simulink subsystem "HEVPowerSplitControl_refsub"  (R2023a)
settings: Solver=VariableStepAuto  StartTime=0.0  StopTime=10.0  RelTol=1e-3
undefined symbols (not defined in the file or in its folder): DiscIntNeverNeededParam, hevcontrol, initial
libraries: simulink x5
settings Model: DefaultTestHarness=HEVPowerSplitControl_refsub_Harness1  Creator=isaacito  LastModifiedBy=isaacito
settings SolverCC: AlgebraicLoopSolver=TrustRegion
settings OptimizationCC: ReuseModelBlockBuffer=off
settings DebuggingCC: UnconnectedInputMsg=warning  UnconnectedOutputMsg=warning  UnconnectedLineMsg=warning
settings ModelReferenceCC: EnableRefExpFcnMdlSchedulingChecks=on
settings RTWCC: DLArmComputeVersion=19.05

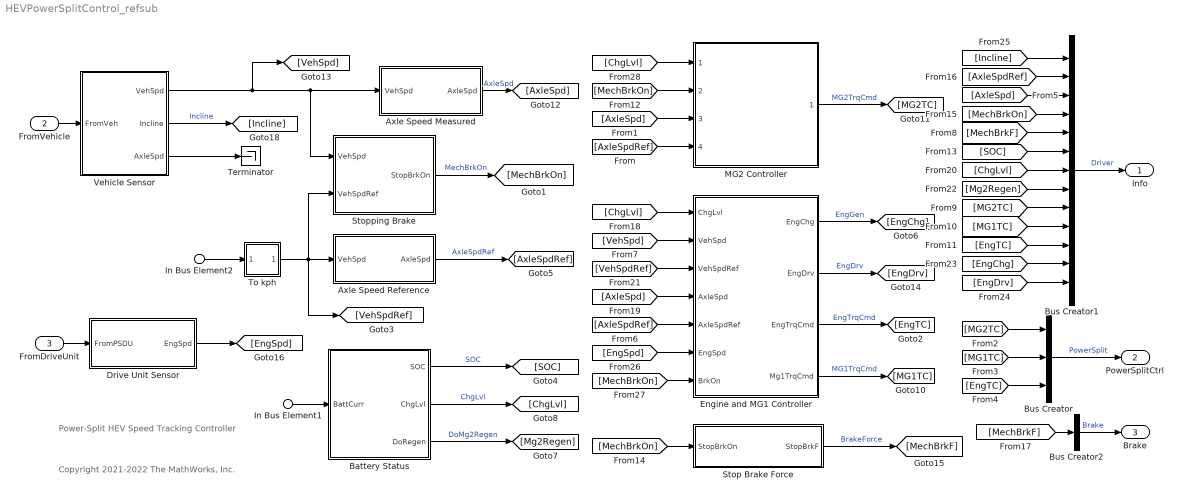
== system HEVPowerSplitControl_refsub ==
  note: Power-Split HEV
      | Speed Tracking Controller
  note: Copyright 2021-2022 The MathWorks, Inc.
  In Bus Element1 : Inport  PortName=FromBattery  Element=Current
  FromVehicle : Inport  Port=2
  FromDriveUnit : Inport  Port=3
  In Bus Element2 : Inport  Port=4  PortName=FromDrvPattern  Element=VehSpdRef
      settings: AttributesFormatString=%<Unit>
  Axle Speed Measured : Subsystem  mask(Vehicle Speed to Axle Speed){Value=hevcontrol.tireRadius_m}
      mask prompts: Value "Tire Rolling Radius [m]"
      mask help: Given longitudinal vehicle speed, this block computes the axle rotational speed.
      mask TypeOptions Value: Tire Rolling Radius (m)/Value
  Axle Speed Reference : Subsystem  mask(Vehicle Speed to Axle Speed){Value=hevcontrol.tireRadius_m}
      mask prompts: Value "Tire Rolling Radius [m]"
      mask help: Given longitudinal vehicle speed, this block computes the axle rotational speed.
      mask TypeOptions Value: Tire Rolling Radius (m)/Value
  Battery Status : Subsystem  mask(Battery Status){capacity_kWh=hevcontrol.hvbattNominalCapacity_kWh, voltagePerCell_V=hevcontrol.hvbattVoltagePerCell_V, initial_SOC_pct=initial.controllerHVBattSOC_pct, SocHigh=hevcontrol.hvbattSocHighMid_pct, SocLow=hevcontrol.hvbattSocMidLow_pct, SocEmpty=hevcontrol.hvbattSocLowEmpty_pct}
      mask prompts: capacity_kWh "Battery Capacity [kW*hr]"; voltagePerCell_V "Voltage per cell [V]"; initial_SOC_pct "Initial SOC [%]"; SocHigh "SOC High-Mid Threshold [%]"; SocLow "SOC Mid-Low Threshold [%]"; SocEmpty "SOC Low-Empty Threshold [%]"
      mask help:
      | Battery current input assumes that the negative (positive) value current means consuming (charging) electric power from (to) the battery.
      |
      | SOC outport outputs the state of charge of the battery in %.
      |
      | ChgLvl outport outputs the charge levels 0 (empty), 1 (low), 2 (mid), or 3 (high). Specify thresholds in SOC Threshold parameters.
      |
      | DoRegen outport outputs true for empty/low/mid battery charge level and false for high. Use this signal to avoid overcharging the battery.
      mask init:
      | if initial_SOC_pct > SocHigh
      |   initialChgLvl = 3;
      | elseif initial_SOC_pct < SocEmpty
      |   initialChgLvl = 0;
      | elseif initial_SOC_pct > SocLow
      |   initialChgLvl = 2;
      | else
      |   initialChgLvl = 1;
      | end
      mask TypeOptions capacity_kWh: SOC Estimation/capacity_kWh
      mask TypeOptions voltagePerCell_V: SOC Estimation/voltagePerCell_V
      mask TypeOptions initial_SOC_pct: SOC Estimation/initial_SOC_pct
      mask DialogControl Container2 Prompt: Parameters
  Bus Creator : BusCreator  Inputs=3
  Bus Creator1 : BusCreator  Inputs=13
  Bus Creator2 : BusCreator  Inputs=1
  Drive Unit Sensor : Subsystem
  Engine and MG1 Controller : Subsystem
  MG2 Controller : Subsystem  ReferencedSubsystem=MG2Controller_HEVPowerSplit_refsub
  Stop Brake Force : Subsystem
  Stopping Brake : Subsystem
  Terminator : Terminator
  To kph : Subsystem
  Vehicle Sensor : Subsystem
  Info : Outport
  PowerSplitCtrl : Outport  Port=2
  Brake : Outport  Port=3
  wires:
  Vehicle Sensor/3(AxleSpd) -> Terminator/1
  In Bus Element2/1 -> To kph/1(In1)
  FromVehicle/1 -> Vehicle Sensor/1(FromVeh)
  Vehicle Sensor/1(VehSpd) -> [VehSpd], Axle Speed Measured/1(VehSpd), Stopping Brake/1(VehSpd)
  Battery Status/1(SOC) -> [SOC]  "SOC"
  [SOC] -> Bus Creator1/6
  [Mg2Regen] -> Bus Creator1/8
  [ChgLvl] -> Bus Creator1/7
  [MechBrkOn] -> Bus Creator1/4
  [AxleSpd] -> Bus Creator1/3
  Engine and MG1 Controller/4(Mg1TrqCmd) -> [MG1TC]  "MG1TrqCmd"
  [VehSpdRef] -> Engine and MG1 Controller/3(VehSpdRef)
  [AxleSpdRef] -> Engine and MG1 Controller/5(AxleSpdRef)
  [AxleSpd] -> Engine and MG1 Controller/4(AxleSpd)
  [AxleSpdRef] -> Bus Creator1/2
  Bus Creator1/1 -> Info/1  "Driver"
  [MG1TC] -> Bus Creator1/10
  [MG2TC] -> Bus Creator1/9
  [MechBrkF] -> Bus Creator1/5
  [EngTC] -> Bus Creator1/11
  [VehSpd] -> Engine and MG1 Controller/2(VehSpd)
  Battery Status/3(DoRegen) -> [Mg2Regen]  "DoMg2Regen"
  Battery Status/2(ChgLvl) -> [ChgLvl]  "ChgLvl"
  Engine and MG1 Controller/3(EngTrqCmd) -> [EngTC]  "EngTrqCmd"
  [ChgLvl] -> Engine and MG1 Controller/1(ChgLvl)
  [EngTC] -> Bus Creator/3
  [MG1TC] -> Bus Creator/2
  [MG2TC] -> Bus Creator/1
  Bus Creator/1 -> PowerSplitCtrl/1  "PowerSplit"
  Axle Speed Reference/1(AxleSpd) -> [AxleSpdRef]  "AxleSpdRef"
  [MechBrkF] -> Bus Creator2/1
  Bus Creator2/1 -> Brake/1  "Brake"
  In Bus Element1/1 -> Battery Status/1(BattCurr)
  Engine and MG1 Controller/1(EngChg) -> [EngChg]  "EngGen"
  Engine and MG1 Controller/2(EngDrv) -> [EngDrv]  "EngDrv"
  [EngChg] -> Bus Creator1/12
  [EngDrv] -> Bus Creator1/13
  [EngSpd] -> Engine and MG1 Controller/6(EngSpd)
  [MechBrkOn] -> Engine and MG1 Controller/7(BrkOn)
  FromDriveUnit/1 -> Drive Unit Sensor/1(FromPSDU)
  Drive Unit Sensor/1(EngSpd) -> [EngSpd]
  [MechBrkOn] -> MG2 Controller/2
  [AxleSpd] -> MG2 Controller/3
  [AxleSpdRef] -> MG2 Controller/4
  [MechBrkOn] -> Stop Brake Force/1(StopBrkOn)
  Vehicle Sensor/2(Incline) -> [Incline]  "Incline"
  MG2 Controller/1 -> [MG2TC]  "MG2TrqCmd"
  Stopping Brake/1(StopBrkOn) -> [MechBrkOn]  "MechBrkOn"
  Stop Brake Force/1(StopBrkF) -> [MechBrkF]  "BrakeForce"
  [Incline] -> Bus Creator1/1
  [ChgLvl] -> MG2 Controller/1
  To kph/1(Out1) -> Axle Speed Reference/1(VehSpd), [VehSpdRef], Stopping Brake/2(VehSpdRef)
  Axle Speed Measured/1(AxleSpd) -> [AxleSpd]  "AxleSpd"

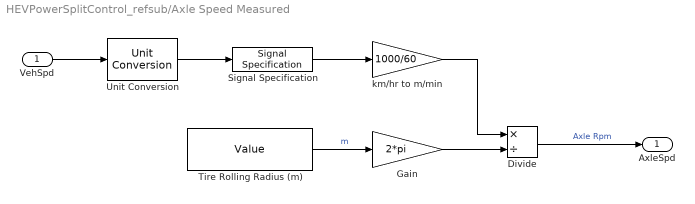
== system HEVPowerSplitControl_refsub/Axle Speed Measured ==
  VehSpd : Inport
      settings: AttributesFormatString=%<Unit>
  Divide : Product  Inputs=*/
  Gain : Gain  Gain=2*pi
  Signal Specification : SignalSpecification  Unit=km/hr
  Tire Rolling Radius (m) : Constant  Value=Value
  Unit Conversion : UnitConversion
  km/hr to m/min : Gain  Gain=1000/60
  AxleSpd : Outport  Unit=rpm  VectorParamsAs1DForOutWhenUnconnected=off
      settings: AttributesFormatString=%<Unit>
  wires:
  km/hr to m/min/1 -> Divide/1
  Signal Specification/1 -> km/hr to m/min/1
  VehSpd/1 -> Unit Conversion/1
  Unit Conversion/1 -> Signal Specification/1
  Divide/1 -> AxleSpd/1  "Axle Rpm"
  Gain/1 -> Divide/2
  Tire Rolling Radius (m)/1 -> Gain/1  "m"

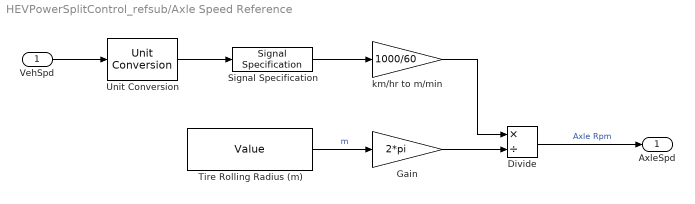
== system HEVPowerSplitControl_refsub/Axle Speed Reference ==
  VehSpd : Inport
      settings: AttributesFormatString=%<Unit>
  Divide : Product  Inputs=*/
  Gain : Gain  Gain=2*pi
  Signal Specification : SignalSpecification  Unit=km/hr
  Tire Rolling Radius (m) : Constant  Value=Value
  Unit Conversion : UnitConversion
  km/hr to m/min : Gain  Gain=1000/60
  AxleSpd : Outport  Unit=rpm  VectorParamsAs1DForOutWhenUnconnected=off
      settings: AttributesFormatString=%<Unit>
  wires:
  km/hr to m/min/1 -> Divide/1
  Signal Specification/1 -> km/hr to m/min/1
  VehSpd/1 -> Unit Conversion/1
  Unit Conversion/1 -> Signal Specification/1
  Divide/1 -> AxleSpd/1  "Axle Rpm"
  Gain/1 -> Divide/2
  Tire Rolling Radius (m)/1 -> Gain/1  "m"

== system HEVPowerSplitControl_refsub/Battery Status ==
  BattCurr : Inport
  Initial Charge Level : InitialCondition  Value=initialChgLvl
  SOC Based States : Stateflow chart  TreatAsAtomicUnit=on
      settings: PortSchema="{\"entries\":[{\"content\":{\"sides\":[{\"content\":{\"connectorIds\":[\"In1\"]},\"type\":\"ConnectorPlacement.EquallySpacedRectSide\",\"uuid\":\"6842a8e0-1533-443f-9239-a32cee073609\"},{\"content\":{\"connectorIds\":[\"Out2\",\"Out1\"],\"side\":\"RIGHT\"},\"type\":\"ConnectorPlacement.EquallySpacedRectSide\",\"uuid\":\"4d5668fa-96aa-414a-86e2-97093b53d80f\"},{\"content\":{\"connectorIds\":[],\"side\":\"TOP\"},\"type\":\"ConnectorPlacement.EquallySpacedRectSide\",\"uuid\":\"b14b12e5-8ddb-4090-8868-1deded7232d1\"},{\"content\":{\"connectorIds\":[],\"side\":\"HIDDEN\"},\"type\":\"ConnectorPlacement.EquallySpacedRectSide\",\"uuid\":\"15641086-7bcd-4523-b266-ad823dacae84\"}]},\"type\":\"ConnectorPlacement.EquallySpacedConnector\",\"uuid\":\"9c75feda-b5f3-44ec-8ad2-652491ceb2eb\"}],\"packageUris\":[\"http://schema.mathworks.com/mf0/Connector/R2020b\"],\"version\":\"1.0\"}"
  SOC Estimation : Subsystem  mask(Battery State-of-Charge Estimation){capacity_kWh=capacity_kWh, voltagePerCell_V=voltagePerCell_V, initial_SOC_pct=initial_SOC_pct}
      mask prompts: capacity_kWh "Battery Capacity [kW*hr]"; voltagePerCell_V "Voltage per cell [V]"; initial_SOC_pct "Initial SOC [%]"
      mask help: Battery current input assumes that the negative value current meas consuming electric power from the battery.
      mask TypeOptions capacity_kWh: Capacity (kW*hr)/Value
      mask TypeOptions voltagePerCell_V: Voltage per Cell (V)/Value
      mask TypeOptions initial_SOC_pct: Initial SOC (%)/Value
  SOC : Outport
  ChgLvl : Outport  Port=2
  DoRegen : Outport  Port=3
  wires:
  Initial Charge Level/1 -> ChgLvl/1
  BattCurr/1 -> SOC Estimation/1(BattCurr)
  SOC Based States/2(BatteryChargeLevel) -> Initial Charge Level/1
  SOC Based States/1(DoRegen) -> DoRegen/1
  SOC Estimation/1(SOC) -> SOC Based States/1(SOC), SOC/1  "SOC"

== system HEVPowerSplitControl_refsub/Drive Unit Sensor ==
  FromPSDU : Inport
  Bus Selector : BusSelector  OutputSignals=eng  OutputAsBus=on
  Bus Selector2 : BusSelector  OutputSignals=EngSpd
  Transfer Fcn : TransferFcn  Denominator=[0.01 1]
  EngSpd : Outport  Unit=rpm
      settings: AttributesFormatString=%<Unit>
  wires:
  Bus Selector/1 -> Bus Selector2/1
  Transfer Fcn/1 -> EngSpd/1
  FromPSDU/1 -> Bus Selector/1
  Bus Selector2/1 -> Transfer Fcn/1  "<EngSpd>"

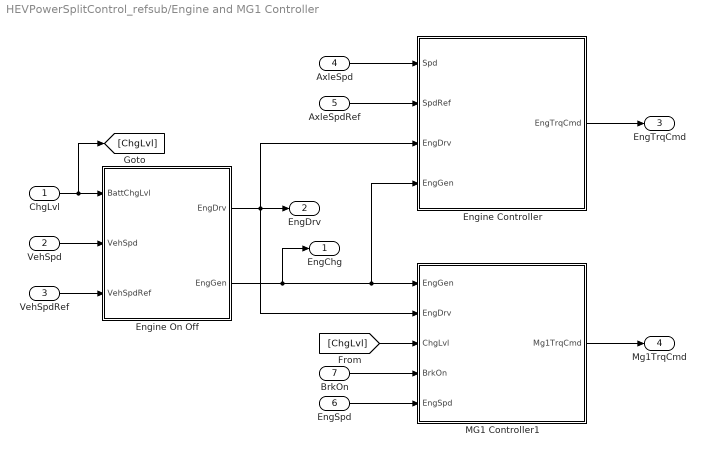
== system HEVPowerSplitControl_refsub/Engine and MG1 Controller ==
  ChgLvl : Inport
  VehSpd : Inport  Port=2  Unit=km/hr
      settings: AttributesFormatString=%<Unit>
  VehSpdRef : Inport  Port=3  Unit=km/hr
      settings: AttributesFormatString=%<Unit>
  AxleSpd : Inport  Port=4  Unit=rpm
      settings: AttributesFormatString=%<Unit>
  AxleSpdRef : Inport  Port=5  Unit=rpm
      settings: AttributesFormatString=%<Unit>
  EngSpd : Inport  Port=6  Unit=rpm
      settings: AttributesFormatString=%<Unit>
  BrkOn : Inport  Port=7
  Engine Controller : Subsystem
  Engine On Off : Stateflow chart  TreatAsAtomicUnit=on
  MG1 Controller1 : Subsystem
  EngChg : Outport
  EngDrv : Outport  Port=2
  EngTrqCmd : Outport  Port=3  Unit=N*m
      settings: AttributesFormatString=%<Unit>
  Mg1TrqCmd : Outport  Port=4  Unit=N*m
      settings: AttributesFormatString=%<Unit>
  wires:
  VehSpd/1 -> Engine On Off/2(VehSpd)
  ChgLvl/1 -> [ChgLvl], Engine On Off/1(BattChgLvl)
  VehSpdRef/1 -> Engine On Off/3(VehSpdRef)
  AxleSpd/1 -> Engine Controller/1(Spd)
  AxleSpdRef/1 -> Engine Controller/2(SpdRef)
  Engine Controller/1(EngTrqCmd) -> EngTrqCmd/1
  BrkOn/1 -> MG1 Controller1/4(BrkOn)
  EngSpd/1 -> MG1 Controller1/5(EngSpd)
  MG1 Controller1/1(Mg1TrqCmd) -> Mg1TrqCmd/1
  [ChgLvl] -> MG1 Controller1/3(ChgLvl)
  Engine On Off/1(EngDrv) -> Engine Controller/3(EngDrv), MG1 Controller1/2(EngDrv), EngDrv/1
  Engine On Off/2(EngGen) -> Engine Controller/4(EngGen), MG1 Controller1/1(EngGen), EngChg/1

== system HEVPowerSplitControl_refsub/Stop Brake Force ==
  StopBrkOn : Inport  OutDataTypeStr=boolean
      settings: AttributesFormatString=%<OutDataTypeStr>
  Brake Force : Subsystem  TreatAsAtomicUnit=on
  Constant1 : Constant  Value=0
  Data Type Conversion : DataTypeConversion  OutDataTypeStr=double  SaturateOnIntegerOverflow=off  RndMeth=Floor
  Hit Crossing : HitCross  HitCrossingOffset=0.5  HitCrossingDirection=rising
      settings: AttributesFormatString=%<HitCrossingOffset>
  Switch : Switch  Criteria=u2 ~= 0  Threshold=0.5  SaturateOnIntegerOverflow=off  InputSameDT=off
  StopBrkF : Outport  Unit=N
      settings: AttributesFormatString=%<Unit>
  wires:
  Data Type Conversion/1 -> Hit Crossing/1
  StopBrkOn/1 -> Data Type Conversion/1, Switch/2
  Hit Crossing/1 -> Brake Force/1(BrakeOnTrigger)
  Brake Force/1(Brake Force) -> Switch/1
  Switch/1 -> StopBrkF/1
  Constant1/1 -> Switch/3

== system HEVPowerSplitControl_refsub/Stopping Brake ==
  VehSpd : Inport
      settings: AttributesFormatString=%<Unit>
  VehSpdRef : Inport  Port=2
      settings: AttributesFormatString=%<Unit>
  Brake On Near Stopping : Stateflow chart  TreatAsAtomicUnit=on
  InitialBrkOn : InitialCondition  Value=initial.driverBrakeOn_tf
  StopBrkOn : Outport  OutDataTypeStr=boolean
      settings: AttributesFormatString=%<OutDataTypeStr>
  wires:
  InitialBrkOn/1 -> StopBrkOn/1
  VehSpdRef/1 -> Brake On Near Stopping/2(VehSpdRef)
  Brake On Near Stopping/1(MechBrkOn) -> InitialBrkOn/1
  VehSpd/1 -> Brake On Near Stopping/1(VehSpd)

== system HEVPowerSplitControl_refsub/To kph ==
  In1 : Inport
  Unit Conversion : UnitConversion
  Out1 : Outport  Unit=km/hr
      settings: AttributesFormatString=%<Unit>
  wires:
  Unit Conversion/1 -> Out1/1
  In1/1 -> Unit Conversion/1

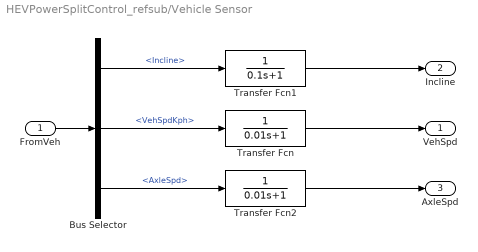
== system HEVPowerSplitControl_refsub/Vehicle Sensor ==
  FromVeh : Inport
  Bus Selector : BusSelector  OutputSignals=Incline,VehSpdKph,AxleSpd
  Transfer Fcn : TransferFcn  Denominator=[0.01 1]
  Transfer Fcn1 : TransferFcn  Denominator=[0.1 1]
  Transfer Fcn2 : TransferFcn  Denominator=[0.01 1]
  VehSpd : Outport  Unit=km/hr
      settings: AttributesFormatString=%<Unit>
  Incline : Outport  Port=2  Unit=deg
      settings: AttributesFormatString=%<Unit>
  AxleSpd : Outport  Port=3  Unit=rpm
      settings: AttributesFormatString=%<Unit>
  wires:
  Bus Selector/3 -> Transfer Fcn2/1  "<AxleSpd>"
  Transfer Fcn1/1 -> Incline/1
  Bus Selector/1 -> Transfer Fcn1/1  "<Incline>"
  Transfer Fcn/1 -> VehSpd/1
  FromVeh/1 -> Bus Selector/1
  Bus Selector/2 -> Transfer Fcn/1  "<VehSpdKph>"
  Transfer Fcn2/1 -> AxleSpd/1

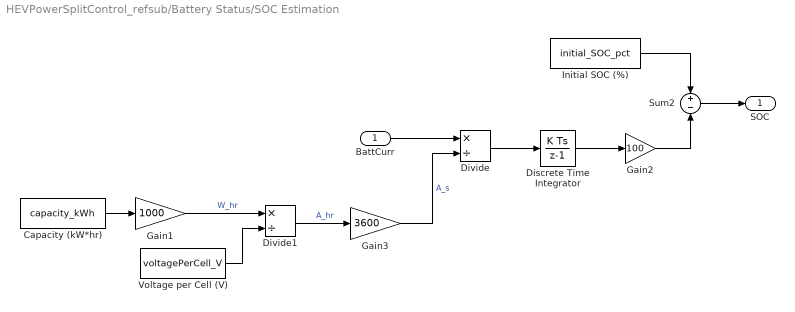
== system HEVPowerSplitControl_refsub/Battery Status/SOC Estimation ==
  BattCurr : Inport  Unit=A
      settings: AttributesFormatString=%<Unit>
  Capacity (kW*hr) : Constant  Value=capacity_kWh
  Discrete Time Integrator : DiscreteIntegrator  SampleTime=-1  ICPrevOutput=DiscIntNeverNeededParam  ICPrevScaledInput=DiscIntNeverNeededParam
  Divide : Product  Inputs=*/
  Divide1 : Product  Inputs=*/
  Gain1 : Gain  Gain=1000
  Gain2 : Gain  Gain=100
  Gain3 : Gain  Gain=3600
  Initial SOC (%) : Constant  Value=initial_SOC_pct
  Sum2 : Sum  Inputs=+-
  Voltage per Cell (V) : Constant  Value=voltagePerCell_V
  SOC : Outport  Unit=%
      settings: AttributesFormatString=%<Unit>
  wires:
  Gain1/1 -> Divide1/1  "W_hr"
  Capacity (kW*hr)/1 -> Gain1/1
  Voltage per Cell (V)/1 -> Divide1/2
  Divide1/1 -> Gain3/1  "A_hr"
  BattCurr/1 -> Divide/1
  Gain3/1 -> Divide/2  "A_s"
  Gain2/1 -> Sum2/2
  Divide/1 -> Discrete Time Integrator/1
  Discrete Time Integrator/1 -> Gain2/1
  Initial SOC (%)/1 -> Sum2/1
  Sum2/1 -> SOC/1

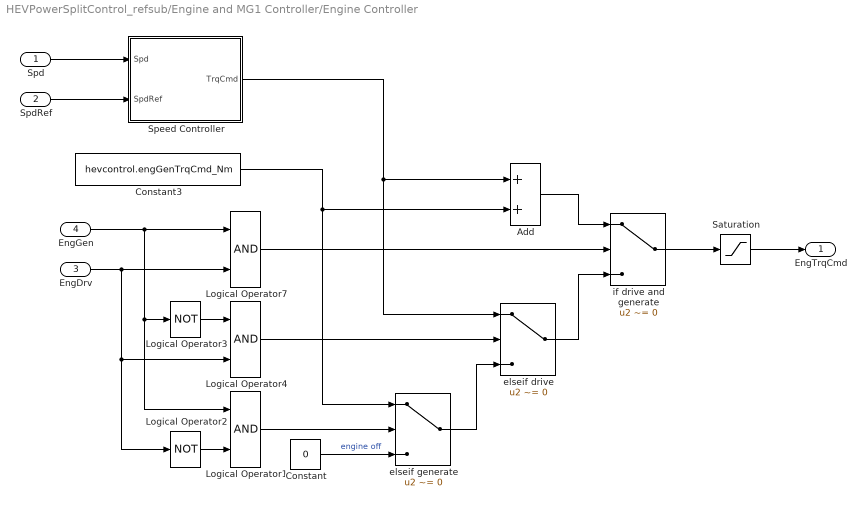
== system HEVPowerSplitControl_refsub/Engine and MG1 Controller/Engine Controller ==
  Spd : Inport  Unit=rpm
      settings: AttributesFormatString=%<Unit>
  SpdRef : Inport  Port=2  Unit=rpm
      settings: AttributesFormatString=%<Unit>
  EngDrv : Inport  Port=3
  EngGen : Inport  Port=4
  Add : Sum
  Constant : Constant  Value=0
  Constant3 : Constant  Value=hevcontrol.engGenTrqCmd_Nm
  Logical Operator1 : Logic  AllPortsSameDT=off  OutDataTypeStr=boolean
  Logical Operator2 : Logic  Operator=NOT  AllPortsSameDT=off  OutDataTypeStr=boolean
  Logical Operator3 : Logic  Operator=NOT  AllPortsSameDT=off  OutDataTypeStr=boolean
  Logical Operator4 : Logic  AllPortsSameDT=off  OutDataTypeStr=boolean
  Logical Operator7 : Logic  AllPortsSameDT=off  OutDataTypeStr=boolean
  Saturation : Saturate  UpperLimit=hevcontrol.engTrqMax_Nm  LowerLimit=0
      settings: AttributesFormatString=|
      | %<UpperLimit>
      | %<LowerLimit>
  Speed Controller : Subsystem
      settings: PortSchema="{\"entries\":[{\"content\":{\"sides\":[{\"content\":{\"connectorIds\":[\"Out1\"]},\"type\":\"ConnectorPlacement.EquallySpacedRectSide\",\"uuid\":\"12b9f2c9-2b28-451b-ad36-7fe4150db485\"},{\"content\":{\"connectorIds\":[\"In1\",\"In2\"],\"side\":\"RIGHT\"},\"type\":\"ConnectorPlacement.EquallySpacedRectSide\",\"uuid\":\"c0fdf9a4-483a-4ddc-b663-6299fcc79327\"},{\"content\":{\"connectorIds\":[],\"side\":\"TOP\"},\"type\":\"ConnectorPlacement.EquallySpacedRectSide\",\"uuid\":\"3f20082e-8487-45e3-9fd7-d6d75741df4d\"}]},\"type\":\"ConnectorPlacement.EquallySpacedConnector\",\"uuid\":\"9361cdd3-74d8-46ee-ae7f-e2dde5d31ed1\"}],\"packageUris\":[\"http://schema.mathworks.com/mf0/Connector/R2020b\"],\"version\":\"1.0\"}"
  elseif drive : Switch  Criteria=u2 ~= 0  SaturateOnIntegerOverflow=off  InputSameDT=off
  elseif generate : Switch  Criteria=u2 ~= 0  SaturateOnIntegerOverflow=off  InputSameDT=off
  if drive and generate : Switch  Criteria=u2 ~= 0  SaturateOnIntegerOverflow=off  InputSameDT=off
  EngTrqCmd : Outport  Unit=N*m
      settings: AttributesFormatString=%<Unit>
  wires:
  if drive and generate/1 -> Saturation/1
  Constant/1 -> elseif generate/3  "engine off"
  elseif generate/1 -> elseif drive/3
  Logical Operator1/1 -> elseif generate/2
  Logical Operator4/1 -> elseif drive/2
  elseif drive/1 -> if drive and generate/3
  Add/1 -> if drive and generate/1
  Logical Operator7/1 -> if drive and generate/2
  Logical Operator3/1 -> Logical Operator4/1
  EngGen/1 -> Logical Operator1/1, Logical Operator3/1, Logical Operator7/1
  Logical Operator2/1 -> Logical Operator1/2
  EngDrv/1 -> Logical Operator7/2, Logical Operator2/1, Logical Operator4/2
  Saturation/1 -> EngTrqCmd/1
  Spd/1 -> Speed Controller/1(Spd)
  SpdRef/1 -> Speed Controller/2(SpdRef)
  Speed Controller/1(TrqCmd) -> Add/1, elseif drive/1
  Constant3/1 -> Add/2, elseif generate/1

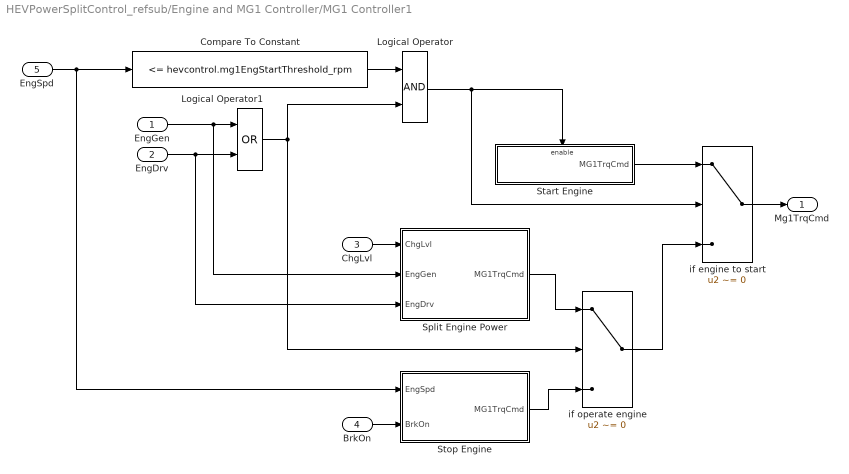
== system HEVPowerSplitControl_refsub/Engine and MG1 Controller/MG1 Controller1 ==
  EngGen : Inport
  EngDrv : Inport  Port=2
  ChgLvl : Inport  Port=3
  BrkOn : Inport  Port=4
  EngSpd : Inport  Port=5  Unit=rpm
      settings: AttributesFormatString=%<Unit>
  Compare To Constant : simulink/Logic and Bit Operations/Compare To Constant  relop=<=  const=hevcontrol.mg1EngStartThreshold_rpm  OutDataTypeStr=boolean
  Logical Operator : Logic  AllPortsSameDT=off  OutDataTypeStr=boolean
  Logical Operator1 : Logic  Operator=OR  AllPortsSameDT=off  OutDataTypeStr=boolean
  Split Engine Power : Subsystem
  Start Engine : Subsystem
  Stop Engine : Subsystem
  if engine to start : Switch  Criteria=u2 ~= 0  SaturateOnIntegerOverflow=off  InputSameDT=off
  if operate engine : Switch  Criteria=u2 ~= 0  SaturateOnIntegerOverflow=off  InputSameDT=off
  Mg1TrqCmd : Outport  Unit=N*m
      settings: AttributesFormatString=%<Unit>
  wires:
  Start Engine/1(MG1TrqCmd) -> if engine to start/1
  if engine to start/1 -> Mg1TrqCmd/1
  if operate engine/1 -> if engine to start/3
  Logical Operator/1 -> Start Engine/Enable, if engine to start/2
  Compare To Constant/1 -> Logical Operator/1
  Split Engine Power/1(MG1TrqCmd) -> if operate engine/1
  ChgLvl/1 -> Split Engine Power/1(ChgLvl)
  Stop Engine/1(MG1TrqCmd) -> if operate engine/3
  EngSpd/1 -> Stop Engine/1(EngSpd), Compare To Constant/1
  BrkOn/1 -> Stop Engine/2(BrkOn)
  Logical Operator1/1 -> Logical Operator/2, if operate engine/2
  EngGen/1 -> Logical Operator1/1, Split Engine Power/2(EngGen)
  EngDrv/1 -> Split Engine Power/3(EngDrv), Logical Operator1/2

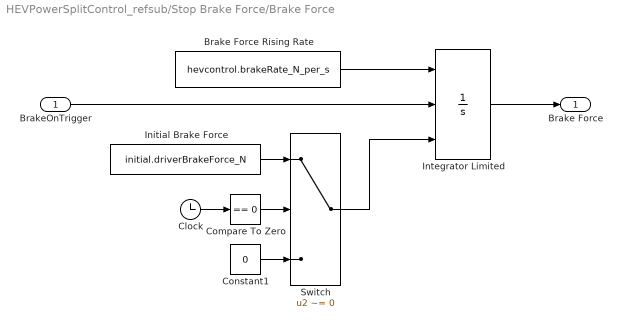
== system HEVPowerSplitControl_refsub/Stop Brake Force/Brake Force ==
  BrakeOnTrigger : Inport
  Brake Force Rising Rate : Constant  Value=hevcontrol.brakeRate_N_per_s
  Clock : Clock
  Compare To Zero : simulink/Logic and Bit Operations/Compare To Zero  relop===  OutDataTypeStr=boolean
  Constant1 : Constant  Value=0
  Initial Brake Force : Constant  Value=initial.driverBrakeForce_N
  Integrator Limited : Integrator  ExternalReset=rising  InitialConditionSource=external  LimitOutput=on  UpperSaturationLimit=hevcontrol.brakeForceMax_N  LowerSaturationLimit=0
      settings: AttributesFormatString=%<UpperSaturationLimit>
  Switch : Switch  Criteria=u2 ~= 0  SaturateOnIntegerOverflow=off  InputSameDT=off
  Brake Force : Outport  Unit=N
      settings: AttributesFormatString=%<Unit>
  wires:
  Brake Force Rising Rate/1 -> Integrator Limited/1
  Constant1/1 -> Switch/3
  Switch/1 -> Integrator Limited/3
  Initial Brake Force/1 -> Switch/1
  Compare To Zero/1 -> Switch/2
  Clock/1 -> Compare To Zero/1
  Integrator Limited/1 -> Brake Force/1
  BrakeOnTrigger/1 -> Integrator Limited/2

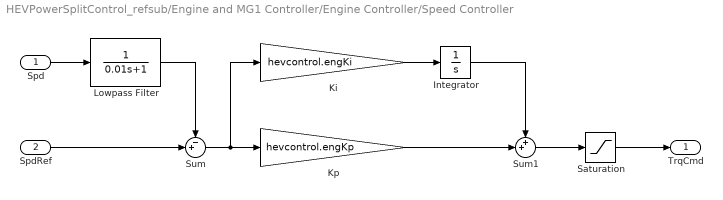
== system HEVPowerSplitControl_refsub/Engine and MG1 Controller/Engine Controller/Speed Controller ==
  Spd : Inport  Unit=rpm
      settings: AttributesFormatString=%<Unit>
  SpdRef : Inport  Port=2  Unit=rpm
      settings: AttributesFormatString=%<Unit>
  Integrator : Integrator  LimitOutput=on  UpperSaturationLimit=hevcontrol.engTrqMax_Nm  LowerSaturationLimit=0
      settings: AttributesFormatString=%<UpperSaturationLimit>
  Ki : Gain  Gain=hevcontrol.engKi
  Kp : Gain  Gain=hevcontrol.engKp
  Lowpass Filter : TransferFcn  Denominator=[0.01 1]
  Saturation : Saturate  UpperLimit=hevcontrol.engTrqMax_Nm  LowerLimit=0
      settings: AttributesFormatString=|
      | %<UpperLimit>
      | %<LowerLimit>
  Sum : Sum  Inputs=-+|
  Sum1 : Sum  Inputs=++|
  TrqCmd : Outport  Unit=N*m  VectorParamsAs1DForOutWhenUnconnected=off
      settings: AttributesFormatString=%<Unit>
  wires:
  SpdRef/1 -> Sum/2
  Spd/1 -> Lowpass Filter/1
  Sum1/1 -> Saturation/1
  Sum/1 -> Ki/1, Kp/1
  Ki/1 -> Integrator/1
  Kp/1 -> Sum1/2
  Integrator/1 -> Sum1/1
  Lowpass Filter/1 -> Sum/1
  Saturation/1 -> TrqCmd/1

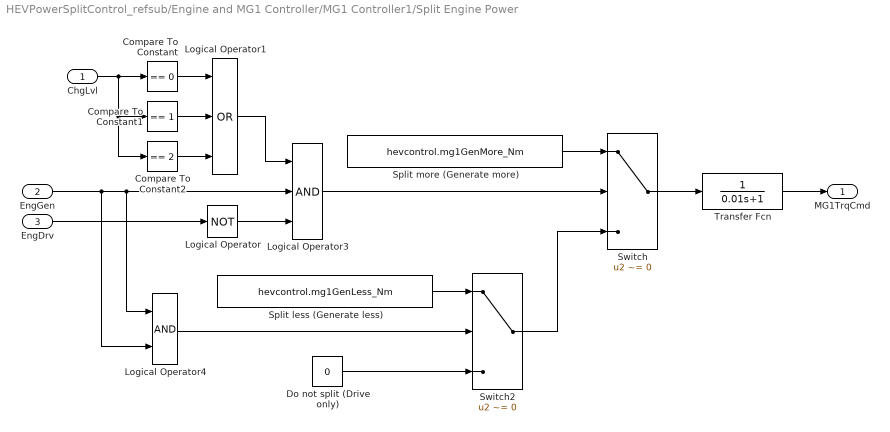
== system HEVPowerSplitControl_refsub/Engine and MG1 Controller/MG1 Controller1/Split Engine Power ==
  ChgLvl : Inport
  EngGen : Inport  Port=2
  EngDrv : Inport  Port=3
  Compare To Constant : simulink/Logic and Bit Operations/Compare To Constant  relop===  const=0  OutDataTypeStr=boolean
  Compare To Constant1 : simulink/Logic and Bit Operations/Compare To Constant  relop===  const=1  OutDataTypeStr=boolean
  Compare To Constant2 : simulink/Logic and Bit Operations/Compare To Constant  relop===  const=2  OutDataTypeStr=boolean
  Do not split (Drive only) : Constant  Value=0
  Logical Operator : Logic  Operator=NOT  Inputs=1  AllPortsSameDT=off  OutDataTypeStr=boolean
  Logical Operator1 : Logic  Operator=OR  Inputs=3  AllPortsSameDT=off  OutDataTypeStr=boolean
  Logical Operator3 : Logic  Inputs=3  AllPortsSameDT=off  OutDataTypeStr=boolean
  Logical Operator4 : Logic  AllPortsSameDT=off  OutDataTypeStr=boolean
  Split less (Generate less) : Constant  Value=hevcontrol.mg1GenLess_Nm
  Split more (Generate more) : Constant  Value=hevcontrol.mg1GenMore_Nm
  Switch : Switch  Criteria=u2 ~= 0  SaturateOnIntegerOverflow=off  InputSameDT=off
  Switch2 : Switch  Criteria=u2 ~= 0  SaturateOnIntegerOverflow=off  InputSameDT=off
  Transfer Fcn : TransferFcn  Denominator=[0.01 1]
  MG1TrqCmd : Outport
  wires:
  Do not split (Drive only)/1 -> Switch2/3
  Split less (Generate less)/1 -> Switch2/1
  Logical Operator4/1 -> Switch2/2
  Switch2/1 -> Switch/3
  Transfer Fcn/1 -> MG1TrqCmd/1
  Logical Operator3/1 -> Switch/2
  Split more (Generate more)/1 -> Switch/1
  Compare To Constant/1 -> Logical Operator1/1
  Logical Operator1/1 -> Logical Operator3/1
  Logical Operator/1 -> Logical Operator3/3
  Compare To Constant2/1 -> Logical Operator1/3
  Compare To Constant1/1 -> Logical Operator1/2
  EngDrv/1 -> Logical Operator/1
  EngGen/1 -> Logical Operator3/2, Logical Operator4/1, Logical Operator4/2
  ChgLvl/1 -> Compare To Constant/1, Compare To Constant1/1, Compare To Constant2/1
  Switch/1 -> Transfer Fcn/1

== system HEVPowerSplitControl_refsub/Engine and MG1 Controller/MG1 Controller1/Start Engine ==
  Enable : EnablePort
  Constant : Constant  Value=hevcontrol.mg1EngStartTrq_Nm
  Transfer Fcn : TransferFcn  Denominator=[0.5 1]
  MG1TrqCmd : Outport  Unit=N*m
      settings: AttributesFormatString=%<Unit>
  wires:
  Transfer Fcn/1 -> MG1TrqCmd/1
  Constant/1 -> Transfer Fcn/1

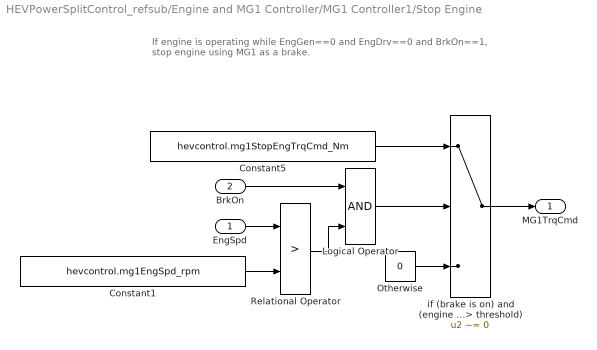
== system HEVPowerSplitControl_refsub/Engine and MG1 Controller/MG1 Controller1/Stop Engine ==
  note: If engine is operating
      | while EngGen==0 and EngDrv==0 and BrkOn==1,
      | stop engine using MG1 as a brake.
  EngSpd : Inport
  BrkOn : Inport  Port=2
  Constant1 : Constant  Value=hevcontrol.mg1EngSpd_rpm
  Constant5 : Constant  Value=hevcontrol.mg1StopEngTrqCmd_Nm
  Logical Operator : Logic  AllPortsSameDT=off  OutDataTypeStr=boolean
  Otherwise : Constant  Value=0
  Relational Operator : RelationalOperator  Operator=>  OutDataTypeStr=boolean  RndMeth=Simplest  InputSameDT=off
  if (brake is on) and (engine speed > threshold) : Switch  Criteria=u2 ~= 0  SaturateOnIntegerOverflow=off  InputSameDT=off
  MG1TrqCmd : Outport
  wires:
  if (brake is on) and (engine speed > threshold)/1 -> MG1TrqCmd/1
  Constant5/1 -> if (brake is on) and (engine speed > threshold)/1
  BrkOn/1 -> Logical Operator/1
  Logical Operator/1 -> if (brake is on) and (engine speed > threshold)/2
  Relational Operator/1 -> Logical Operator/2
  EngSpd/1 -> Relational Operator/1
  Otherwise/1 -> if (brake is on) and (engine speed > threshold)/3
  Constant1/1 -> Relational Operator/2

== stateflow chart HEVPowerSplitControl_refsub/Engine and MG1 Controller/Engine On Off ==
  state Initial
  state EngineOff
    entry:
    EngDrv = false;
    EngGen = false;
  state EngineDriveGenerate
    entry:
    EngDrv = true;
    EngGen = true;
  state EngineDrive
    entry:
    EngDrv = true;
    EngGen = false;
  state EngineGenerate
    entry:
    EngDrv = false;
    EngGen = true;
  (default) -> Initial
  Initial -> (junction 34) [order 2] : [ (BattChgLvl == 2 || BattChgLvl == 3) ...
      |  && VehSpdRef < engOnVehSpd ]
  Initial -> (junction 36) [order 1] : [ BattChgLvl == 1 ...
      |  && 0.01 < VehSpdRef ]
  (junction 34) -> EngineOff
  (junction 36) -> EngineDriveGenerate
  Initial -> (junction 42) [order 4] : [ (BattChgLvl == 2 || BattChgLvl == 3) ...
      |  && engOnVehSpd <= VehSpdRef ]
  (junction 42) -> EngineDrive
  Initial -> EngineGenerate [order 3] : [ BattChgLvl == 0 ...
      |   || (BattChgLvl == 1 ...
      |        && VehSpdRef < 0.01) ]
  (junction 30) -> EngineOff
  EngineDriveGenerate -> (junction 30) [order 3] : [ BattChgLvl == 3 ...
      |  && VehSpd < engOnVehSpd - 10 ]
  (junction 50) -> EngineOff : [ (BattChgLvl == 2 || BattChgLvl == 3) ...
      |   && VehSpd < engOnVehSpd - 10 ]
  EngineDrive -> (junction 50) [order 1]
  EngineOff -> (junction 54) [order 1]
  (junction 46) -> EngineOff
  EngineOff -> (junction 44) [order 2] : [ (BattChgLvl == 0 ...
      |     || BattChgLvl == 1) ...
      |  || (BattChgLvl == 2 ...
      |      && chgSpd < VehSpd) ]
  (junction 54) -> EngineDrive : [ (BattChgLvl == 2 || BattChgLvl == 3) ...
      |   && engOnVehSpd < VehSpd ...
      |   && VehSpd < VehSpdRef + 0.1 ]
  EngineDriveGenerate -> EngineDrive [order 2] : [ BattChgLvl == 3 ...
      | && engOnVehSpd - 10 < VehSpd ]
  EngineDrive -> EngineDriveGenerate [order 2] : [ BattChgLvl == 1 ...
      | || (BattChgLvl == 2 ...
      |      && chgSpd < VehSpd) ]
  (junction 38) -> EngineDriveGenerate
  EngineDriveGenerate -> (junction 40) [order 1] : [ BattChgLvl == 0 ...
      | || ((BattChgLvl == 1 || BattChgLvl == 2) ...
      |      && abs(VehSpd) < 0.01) ]
  (junction 48) -> EngineDrive
  (junction 40) -> EngineGenerate
  EngineGenerate -> (junction 48) [order 1] : [ BattChgLvl == 3 ...
      |  && engOnVehSpd < VehSpd ]
  EngineGenerate -> (junction 46) [order 2] : [ BattChgLvl == 3 ...
      |  && VehSpd < engOnVehSpd ]
  EngineGenerate -> (junction 38) [order 3] : [ (BattChgLvl == 1 || BattChgLvl == 2) ...
      |  && 1 < VehSpdRef ]
  (junction 44) -> EngineGenerate
  data: BattChgLvl input; VehSpd input; engOnVehSpd local double =hevcontrol.engOnVehSpd_kph; EngDrv output; VehSpdRef input; chgSpd local double =hevcontrol.chgSpd_kph; EngGen output

== stateflow chart HEVPowerSplitControl_refsub/Stopping Brake/Brake On Near Stopping ==
  state Initial
  state BrakeOn
    entry:
    MechBrkOn = true;
  state BrakeOff
    entry:
    MechBrkOn = false;
  (default) -> Initial
  Initial -> (junction 22) [order 2] : [abs(VehSpd) <= BrkOnSpd]
  Initial -> (junction 24) [order 1] : [ BrkOnSpd < VehSpd ...
      |  || VehSpd < -BrkOnSpd]
  (junction 22) -> BrakeOn
  (junction 24) -> BrakeOff
  BrakeOn -> BrakeOff : [ VehSpdRef > 0.01 ...
      |  && (BrkOffDeltaSpd < VehSpdRef - VehSpd...
      |       || VehSpdRef - VehSpd < -BrkOffDeltaSpd ) ]
  BrakeOff -> BrakeOn : [ abs(VehSpd) < BrkOnSpd ...
      |  && abs(VehSpdRef) < 0.001 ]
  data: VehSpd input; MechBrkOn output; VehSpdRef input; BrkOnSpd local double =hevcontrol.brakeOnSpd_kph; BrkOffDeltaSpd local double =hevcontrol.brakeOffSpdDiff_kph

== stateflow chart HEVPowerSplitControl_refsub/Battery Status/SOC Based States ==
  state SocHigh
    entry:
    BatteryChargeLevel = 3;
    DoRegen = false;
  state Classify
  state SocOk
    entry:
    BatteryChargeLevel = 2;
    DoRegen = true;
  state SocLow
    entry:
    BatteryChargeLevel = 1;
    DoRegen = true;
  state SocEmpty
    entry:
    BatteryChargeLevel = 0;
    DoRegen = true;
  (junction 11) -> SocHigh : [ SocHigh <= SOC ]
  Classify -> (junction 11) [order 1]
  SocOk -> SocHigh [order 1] : [ SocHigh + 2 < SOC ]
  SocHigh -> SocOk : [ SOC < SocHigh - 2 ]
  Classify -> SocOk [order 2] : [ SocLow <= SOC & SOC < SocHigh ]
  (default) -> Classify
  Classify -> (junction 31) [order 4]
  Classify -> (junction 15) [order 3]
  SocLow -> SocOk [order 1] : [ SocLow + 2 < SOC ]
  SocOk -> SocLow [order 2] : [ SOC < SocLow - 2 ]
  (junction 15) -> SocLow : [ SocEmpty <= SOC & SOC < SocLow ]
  SocEmpty -> SocLow : [ SocEmpty + 1 < SOC ]
  SocLow -> SocEmpty [order 2] : [ SOC < SocEmpty - 1 ]
  (junction 31) -> SocEmpty : [ SOC < SocEmpty ]
  data: SOC input; SocLow parameter double; SocHigh parameter double; DoRegen output; BatteryChargeLevel output; SocEmpty parameter
